simulink model "dc_motor_lls"  (R2026a)
settings: Solver=FixedStepDiscrete  StopTime=T_exp  FixedStep=Ts  EnableMultiTasking=on
model workspace (MATLAB code in the model file):
  | % Parameters for this model (edit here, then press Ctrl+D to update)
  | Ts = 0.01;              % sample time [s]
  | T_exp = 60;             % length of the experiment [s]
  | Vs = 6;                 % maximum motor voltage (motor rating) [V]
  | CPR = 12*298;           % encoder counts per output-shaft revolution
  | 
  | % Open-loop excitation: offset + two square waves (PWM duty, 0-255)
  | % (duty varies between pwm_offset - pwm_amp1 - pwm_amp2 and
  | %  pwm_offset + pwm_amp1 + pwm_amp2; keep the minimum above the dead-band)
  | pwm_offset = 140;       % mean duty
  | pwm_amp1 = 50;  per1 = 3.0;   % square wave 1: amplitude, period [s]
  | pwm_amp2 = 30;  per2 = 7.4;   % square wave 2: amplitude, period [s]
  | V_supply = 6;            % driver supply voltage [V] (hardware value set below)
  | t_start = 1;            % excitation starts at [s]
  | 
  | % Speed low-pass filter (also applied to the voltage for estimation)
  | filt_num = 0.2;  filt_den = [1 -0.8];
  | 
  | % Estimator
  | D = 5;                  % estimate every D samples (Te = D*Ts)
  | NMin = 20;              % estimation steps before the first estimate
  | 
  | % Hardware: Cytron Maker Drive from a 9 V battery, 6 V motor
  | V_supply = 9;           % driver supply voltage [V] (PWM duty 255 = V_supply)
  | pwm_offset = 150;  pwm_amp1 = 15;  pwm_amp2 = 5;   % duty 130-170, i.e. 4.6-6 V (above the motor's sticking region)
libraries: arduinosensorlib x1, arduinolib x1
settings Model: SimulationMode=external  SILPILModeSetting=veronly  ExtModeTrigDuration=2  Creator=00782620  LastModifiedBy=00782620
settings HardwareCC: ProdBitPerInt=16.0  ProdBitPerPointer=16.0  ProdBitPerSizeT=16.0  ProdBitPerPtrDiffT=16.0  ProdWordSize=8.0  ProdHWDeviceType=Atmel->AVR
settings RTWCC: SystemTargetFile=ert.tlc  HardwareBoard=Arduino Mega 2560  TLCOptions=-aInlineSetEventsForThisBaseRateFcn=TLC_FALSE -aSuppressMultiTaskScheduler=TLC_FALSE -aRateBasedStepFcn=1  Toolchain=Arduino AVR  BuildConfiguration=Faster Runs  Description=Embedded Coder
settings ERTTargetCC: ExtModeTransport=3.0  ExtModeAutomaticAllocSize=off  ExtModeStaticAllocSize=2048.0  SupportContinuousTime=on  SupportVariableSizeSignals=on

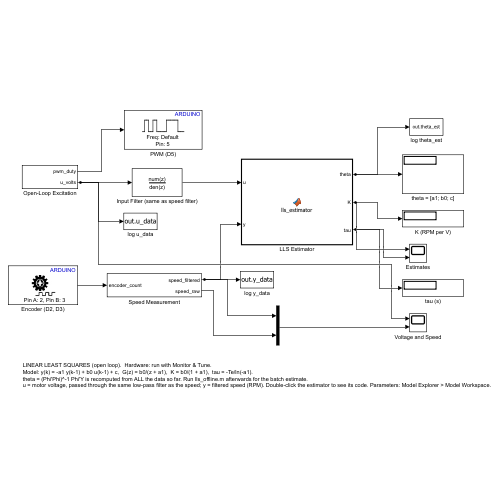
[thumbnail: Simulink's stored preview of the top-level diagram]
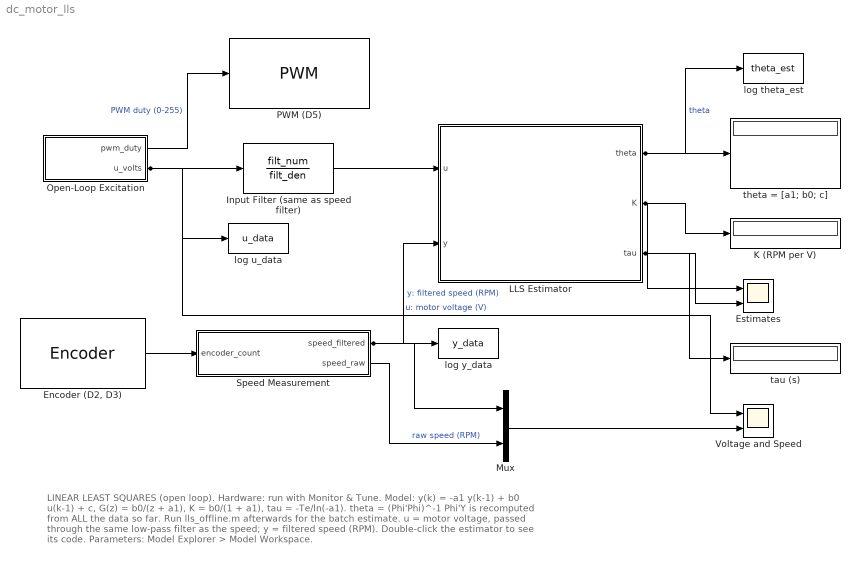
== system dc_motor_lls ==
  note: LINEAR LEAST SQUARES (open loop).  Hardware: run with Monitor & Tune.
      | Model: y(k) = -a1 y(k-1) + b0 u(k-1) + c,  G(z) = b0/(z + a1),  K = b0/(1 + a1),  tau = -Te/ln(-a1).
      | theta = (Phi'Phi)^-1 Phi'Y is recomputed from ALL the data so far. Run lls_offline.m afterwards for the batch estimate.
      | u = motor voltage, passed through the same low-pass filter as the speed; y = filtered speed (RPM). Double-click the estimator to see its code. Parameters: Model Explorer > Model Workspace.
  "Encoder (D2, D3)" : arduinosensorlib/Encoder  InputA=2  InputB=3  Mode=No reset  SampleTime=Ts
  Estimates : Scope  NumInputPorts=2
  Input Filter (same as speed filter) : DiscreteFilter  Numerator=filt_num  Denominator=filt_den  SampleTime=Ts
  K (RPM per V) : Display
  LLS Estimator : MATLAB Function  TreatAsAtomicUnit=on
  Mux : Mux  Inputs=2
  Open-Loop Excitation : Subsystem
  PWM (D5) : arduinolib/PWM  pinNumber=5  frequencyType=Default  desiredFrequency=490.2  achievableFrequency=490.2
  Speed Measurement : Subsystem
  Voltage and Speed : Scope  NumInputPorts=2
  log theta_est : ToWorkspace  VariableName=theta_est  SampleTime=-1
  log u_data : ToWorkspace  VariableName=u_data  SampleTime=-1
  log y_data : ToWorkspace  VariableName=y_data  SampleTime=-1
  tau (s) : Display
  theta = [a1; b0; c] : Display
  wires:
  Open-Loop Excitation/1(pwm_duty) -> PWM (D5)/1  "PWM duty (0-255)"
  Speed Measurement/2(speed_raw) -> Mux/2  "raw speed (RPM)"
  Open-Loop Excitation/2(u_volts) -> Input Filter (same as speed filter)/1, log u_data/1, Voltage and Speed/1  "u: motor voltage (V)"
  LLS Estimator/3(tau) -> tau (s)/1, Estimates/2
  "Encoder (D2, D3)"/1 -> Speed Measurement/1(encoder_count)
  LLS Estimator/2(K) -> K (RPM per V)/1, Estimates/1
  Input Filter (same as speed filter)/1 -> LLS Estimator/1(u)
  Speed Measurement/1(speed_filtered) -> log y_data/1, Mux/1, LLS Estimator/2(y)  "y: filtered speed (RPM)"
  LLS Estimator/1(theta) -> theta = [a1; b0; c]/1, log theta_est/1  "theta"
  Mux/1 -> Voltage and Speed/2

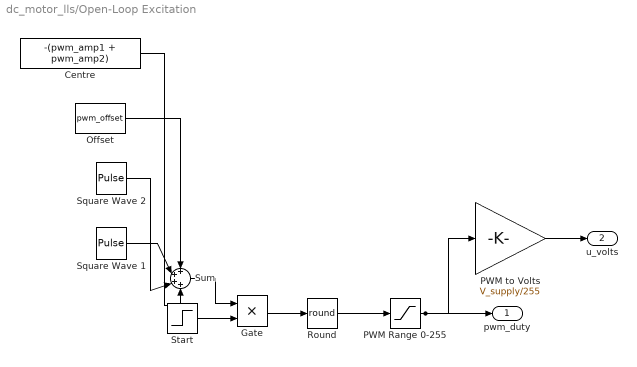
== system dc_motor_lls/Open-Loop Excitation ==
  Centre : Constant  Value=-(pwm_amp1 + pwm_amp2)  SampleTime=Ts
  Gate : Product
  Offset : Constant  Value=pwm_offset  SampleTime=Ts
  PWM Range 0-255 : Saturate  UpperLimit=floor(255*Vs/V_supply)  LowerLimit=0
  PWM to Volts : Gain  Gain=V_supply/255
  Round : Rounding  Operator=round
  Square Wave 1 : DiscretePulseGenerator  Amplitude=2*pwm_amp1  Period=round(per1/Ts)  PulseWidth=round(per1/Ts/2)  SampleTime=Ts
  Square Wave 2 : DiscretePulseGenerator  Amplitude=2*pwm_amp2  Period=round(per2/Ts)  PulseWidth=round(per2/Ts/2)  SampleTime=Ts
  Start : Step  Time=t_start  SampleTime=Ts
  Sum : Sum  Inputs=++++
  pwm_duty : Outport
  u_volts : Outport  Port=2
  wires:
  Centre/1 -> Sum/4
  Start/1 -> Gate/2
  Offset/1 -> Sum/1
  Gate/1 -> Round/1
  Square Wave 2/1 -> Sum/3
  Square Wave 1/1 -> Sum/2
  Sum/1 -> Gate/1
  Round/1 -> PWM Range 0-255/1
  PWM Range 0-255/1 -> PWM to Volts/1, pwm_duty/1
  PWM to Volts/1 -> u_volts/1

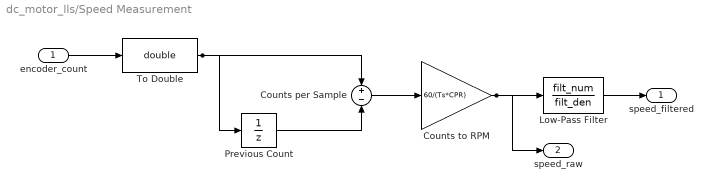
== system dc_motor_lls/Speed Measurement ==
  encoder_count : Inport
  Counts per Sample : Sum  Inputs=+-
  Counts to RPM : Gain  Gain=60/(Ts*CPR)
  Low-Pass Filter : DiscreteFilter  Numerator=filt_num  Denominator=filt_den  SampleTime=Ts
  Previous Count : UnitDelay  SampleTime=Ts
  To Double : DataTypeConversion  OutDataTypeStr=double  SaturateOnIntegerOverflow=off  RndMeth=Floor
  speed_filtered : Outport
  speed_raw : Outport  Port=2
  wires:
  Counts per Sample/1 -> Counts to RPM/1
  encoder_count/1 -> To Double/1
  To Double/1 -> Counts per Sample/1, Previous Count/1
  Low-Pass Filter/1 -> speed_filtered/1
  Previous Count/1 -> Counts per Sample/2
  Counts to RPM/1 -> Low-Pass Filter/1, speed_raw/1

== matlab function dc_motor_lls/LLS Estimator ==
  data: u input; theta output; y input; K output; tau output; Ts parameter; D parameter; t_start parameter; NMin parameter
function [theta, K, tau] = lls_estimator(u, y, Ts, D, t_start, NMin)
% Linear least squares (LLS) estimate of a first-order DC motor model
%
%   y(k) = -a1*y(k-1) + b0*u(k-1) + c,    theta = [a1; b0; c]
%
%   G(z) = b0/(z + a1),  K = b0/(1 + a1),  tau = -Te/ln(-a1)
%   c is a constant term that accounts for the motor dead-band (friction).
%
%   theta = (Phi'*Phi) \ (Phi'*Y), where each row of Phi is
%   phi' = [-y(k-1), u(k-1), 1]. Phi'*Phi and Phi'*Y are accumulated one
%   step at a time, so theta is the batch LLS solution using ALL of the data
%   collected so far (every sample weighted equally).
%
%   u     motor voltage [V] (passed through the same filter as the speed)
%   y     filtered motor speed [RPM]
%   Ts    sample time [s];  D: estimate every D samples, Te = D*Ts
%   t_start  time the excitation starts [s] (earlier data are not used)
%   NMin  number of estimation steps before the first estimate

persistent PhiTPhi PhiTY N count uSum yPrev th k
if isempty(PhiTPhi)
    PhiTPhi = zeros(3, 3);     % running sum of phi*phi'
    PhiTY = zeros(3, 1);       % running sum of phi*y
    N = 0;                     % number of estimation steps
    count = D - 1;             % first estimation step at k = 0
    uSum = 0;                  % sum of u over the current interval
    yPrev = 0;                 % y at the previous estimation step
    th = zeros(3, 1);          % estimate [a1; b0; c]
    k = 0;                     % sample number
end
u = double(u);
y = double(y);
k = k + 1;

count = count + 1;
if count >= D
    uAvg = uSum/D;                       % average input over the interval
    phi = [-yPrev; uAvg; 1];             % regressor
    if (k - D)*Ts >= t_start             % only use data after the start
        PhiTPhi = PhiTPhi + phi*phi';    % accumulate Phi'*Phi
        PhiTY = PhiTY + phi*y;           % accumulate Phi'*Y
        N = N + 1;
    end
    if N >= NMin && rcond(PhiTPhi) > 1e-12
        th = PhiTPhi \ PhiTY;            % solve the normal equations
    end
    yPrev = y;
    uSum = u;                            % start the next interval
    count = 0;
else
    uSum = uSum + u;
end

theta = th;
[K, tau] = firstOrderParams(th, D*Ts);
end

function [K, tau] = firstOrderParams(th, Te)
% Gain and time constant of G(z) = b0/(z + a1), sampled at Te
K = 0;
tau = 0;
if abs(1 + th(1)) > 1e-9
    K = th(2)/(1 + th(1));
end
p = -th(1);                              % pole of the discrete-time model
if p > 0 && p < 1
    tau = -Te/log(p);
end
end
